simulink model "b0_closed"  (R2023b)
settings: Solver=FixedStepDiscrete  StartTime=0.0  StopTime=60  FixedStep=0.001  RelTol=1e-3
undefined symbols (not defined in the file or in its folder): DiscIntNeverNeededParam
settings Model: Creator=28447  LastModifiedBy=28447
settings SFSimCC: SimUserIncludeDirs=D:\Desktop\RCESO\simulink
settings SFSimCC: SimCustomHeaderCode=|
  | typedef struct { float b0; float du; } b0_res_t;
  | extern b0_res_t b0_ident_res(float iq, float u, float omega, float e1, float v);
settings SFSimCC: SimUserSources=|
  | D:\Desktop\RCESO\simulink\b0_ident.c
  | D:\Desktop\RCESO\simulink\b0_ident_wrap.c

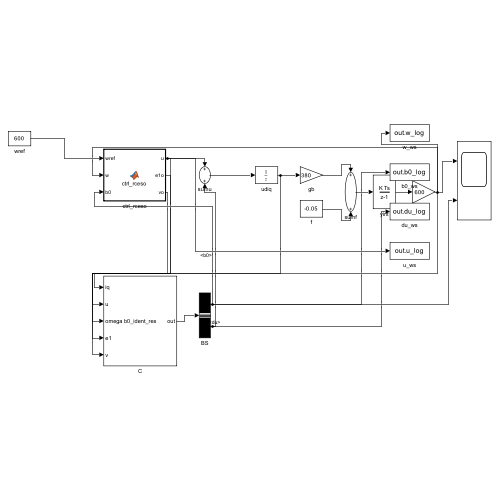
[thumbnail: Simulink's stored preview of the top-level diagram]
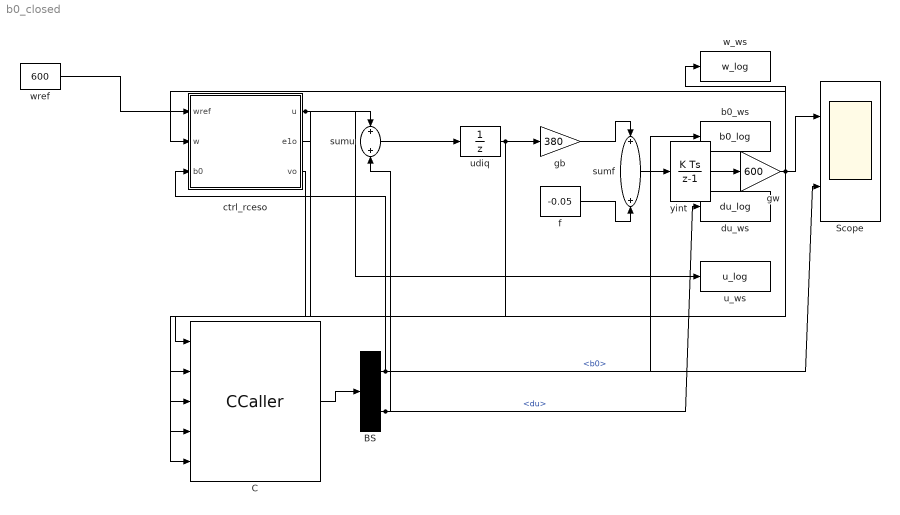
== system b0_closed ==
  BS : BusSelector  OutputSignals=b0,du
  C : CCaller  FunctionName=b0_ident_res  PortSpecificationStruct="%)30     .    4 H   8    (     @         %    \"     8    !     0         %  0 \"0    $    _    07)G3F%M90  4&]R=$YA;64 4V-O<&4     26YD97@     5'EP90      4VEZ90      27-';&]B86P   X    P    !@    @    $          4    (     0    ,    !         !   P!O=70 #@   #     &    \"     0         !0    @    !     P    $         $  # &]U=  .    .     8    (    !          %    \"     $    &     0         0   ...(+3175 chars)"
  Scope : Scope  NumInputPorts=2
  b0_ws : ToWorkspace  VariableName=b0_log  SaveFormat=Timeseries  SampleTime=0.001
  ctrl_rceso : MATLAB Function  TreatAsAtomicUnit=on
  du_ws : ToWorkspace  VariableName=du_log  SaveFormat=Timeseries  SampleTime=0.001
  f : Constant  Value=-0.05  OutDataTypeStr=single  SampleTime=0.001
  gb : Gain  Gain=380  OutDataTypeStr=single
  gw : Gain  Gain=600  OutDataTypeStr=single
  sumf : Sum  OutDataTypeStr=single
  sumu : Sum  OutDataTypeStr=single
  u_ws : ToWorkspace  VariableName=u_log  SaveFormat=Timeseries  SampleTime=0.001
  udiq : UnitDelay  SampleTime=0.001  HasFrameUpgradeWarning=on
  w_ws : ToWorkspace  VariableName=w_log  SaveFormat=Timeseries  SampleTime=0.001
  wref : Constant  Value=600  OutDataTypeStr=single  SampleTime=0.001
  yint : DiscreteIntegrator  SampleTime=0.001  OutDataTypeStr=single  ICPrevOutput=DiscIntNeverNeededParam  ICPrevScaledInput=DiscIntNeverNeededParam
  wires:
  wref/1 -> ctrl_rceso/1(wref)
  ctrl_rceso/1(u) -> sumu/1, C/2, u_ws/1
  BS/2 -> sumu/2, du_ws/1  "<du>"
  sumu/1 -> udiq/1
  udiq/1 -> gb/1, C/1
  gb/1 -> sumf/1
  f/1 -> sumf/2
  sumf/1 -> yint/1
  yint/1 -> gw/1
  gw/1 -> ctrl_rceso/2(w), C/3, w_ws/1, Scope/1
  BS/1 -> ctrl_rceso/3(b0), b0_ws/1, Scope/2  "<b0>"
  ctrl_rceso/2(e1o) -> C/4
  ctrl_rceso/3(vo) -> C/5
  C/1 -> BS/1

== matlab function b0_closed/ctrl_rceso ==
  data: wref input; u output; w input; b0 input; e1o output; vo output
function [u, e1o, vo] = ctrl_rceso(wref, w, b0)
%#codegen
persistent init z1 z2 v vbuf vi uprev
if isempty(init)
    init = 1; z1 = 0; z2 = 0; v = 0; vbuf = zeros(1,50); vi = 1; uprev = 0;
end
dt = 1e-3;
kp = 75.36; wo = 500; b3 = 4000; zeta = 0.2; tau0 = 20e-3; Q0 = 0.98;
yref = wref/600;
e1 = yref - z1;
vd = vbuf(vi);
vchi = Q0*vd + b3*tanh(e1/zeta);
vn = vchi + (v - vchi)*exp(-dt/tau0);
vbuf(vi) = v; vi = vi+1; if vi > 50, vi = 1; end
z1n = z1 + dt*(z2 + b0*uprev + v + 2*wo*e1);
z2n = z2 + dt*(wo*wo*e1);
en = yref - z1n;
u = (kp*en - z2n - vn)/b0;
z1 = z1n; z2 = z2n; v = vn; uprev = u;
e1o = e1; vo = vn;
% 与 Simulink 全 single 模型一致
u = single(u); e1o = single(e1o); vo = single(vo);
end
